simulink model "longitudinal_L1"  (R2023b)
settings: Solver=ode45  StartTime=0.0  StopTime=scn.t_end  MaxStep=0.01  RelTol=1e-3
undefined symbols (not defined in the file): bat, lim, scn, thr, veh
settings Model: Creator=Pol Cruañas  LastModifiedBy=Pol Cruañas

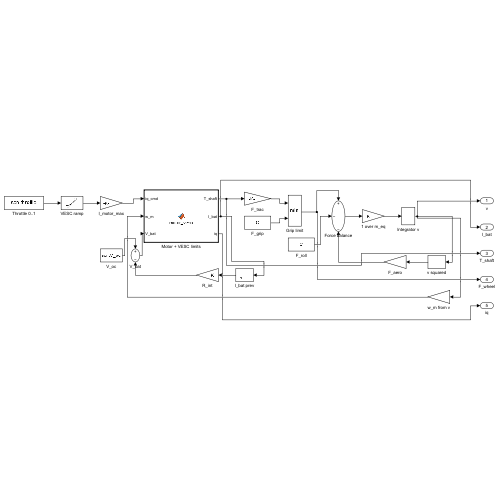
[thumbnail: Simulink's stored preview of the top-level diagram]
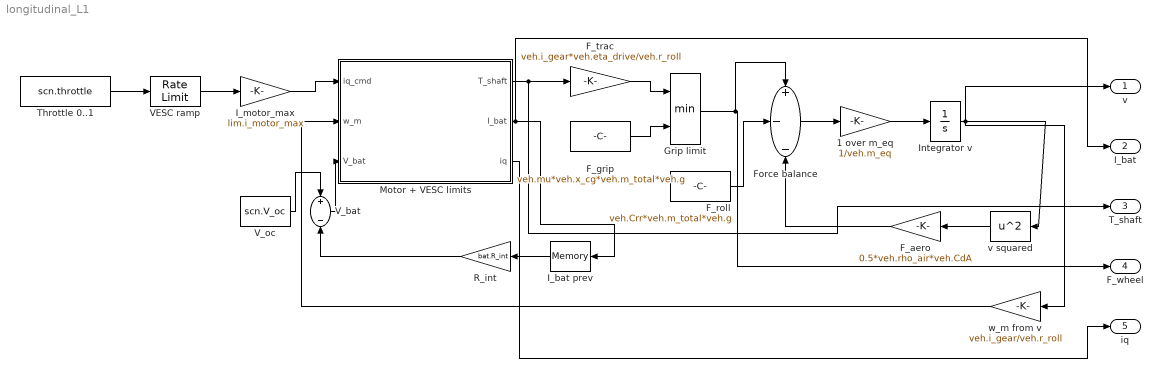
== system longitudinal_L1 ==
  1 over m_eq : Gain  Gain=1/veh.m_eq
  F_aero : Gain  Gain=0.5*veh.rho_air*veh.CdA
  F_grip : Constant  Value=veh.mu*veh.x_cg*veh.m_total*veh.g
  F_roll : Constant  Value=veh.Crr*veh.m_total*veh.g
  F_trac : Gain  Gain=veh.i_gear*veh.eta_drive/veh.r_roll
  Force balance : Sum  Inputs=+--
  Grip limit : MinMax  Inputs=2
  I_bat prev : Memory
  I_motor_max : Gain  Gain=lim.i_motor_max
  Integrator v : Integrator  InitialCondition=scn.v0  LimitOutput=on  LowerSaturationLimit=0
  Motor + VESC limits : MATLAB Function  TreatAsAtomicUnit=on
  R_int : Gain  Gain=bat.R_int
  Throttle 0..1 : FromWorkspace  VariableName=scn.throttle
  VESC ramp : RateLimiter  RisingSlewLimit=1/thr.ramp_time_pos  FallingSlewLimit=-1/thr.ramp_time_neg  SampleTimeMode=inherited
  V_bat : Sum  Inputs=+-
  V_oc : Constant  Value=scn.V_oc
  v squared : Math  Operator=square
  w_m from v : Gain  Gain=veh.i_gear/veh.r_roll
  v : Outport
  I_bat : Outport  Port=2
  T_shaft : Outport  Port=3
  F_wheel : Outport  Port=4
  iq : Outport  Port=5
  wires:
  Throttle 0..1/1 -> VESC ramp/1
  VESC ramp/1 -> I_motor_max/1
  I_motor_max/1 -> Motor + VESC limits/1(iq_cmd)
  w_m from v/1 -> Motor + VESC limits/2(w_m)
  V_bat/1 -> Motor + VESC limits/3(V_bat)
  Motor + VESC limits/1(T_shaft) -> F_trac/1, T_shaft/1
  Motor + VESC limits/2(I_bat) -> I_bat prev/1, I_bat/1
  I_bat prev/1 -> R_int/1
  V_oc/1 -> V_bat/1
  R_int/1 -> V_bat/2
  F_trac/1 -> Grip limit/1
  F_grip/1 -> Grip limit/2
  Grip limit/1 -> Force balance/1, F_wheel/1
  F_roll/1 -> Force balance/2
  F_aero/1 -> Force balance/3
  Force balance/1 -> 1 over m_eq/1
  1 over m_eq/1 -> Integrator v/1
  Integrator v/1 -> v squared/1, w_m from v/1, v/1
  v squared/1 -> F_aero/1
  Motor + VESC limits/3(iq) -> iq/1

== matlab function longitudinal_L1/Motor + VESC limits ==
  data: iq_cmd input; T_shaft output; w_m input; V_bat input; I_bat output; iq output; P parameter
function [T_shaft, I_bat, iq] = motor_vesc(iq_cmd, w_m, V_bat, P)
% Quasi-static PMSM with id = 0 and the three VESC limits on iq.
we = P.p * w_m;                                % electrical speed [rad/s]
Vmax = P.duty_max * V_bat / sqrt(3);           % SVPWM voltage ceiling
% 1) Voltage limit: |v_dq| = Vmax, vd = -we*Lq*iq, vq = R*iq + we*lambda
a  = P.Rs^2 + (we*P.Lq)^2;
bq = 2*P.Rs*we*P.lambda;
c  = (we*P.lambda)^2 - Vmax^2;
disc = bq^2 - 4*a*c;
if disc > 0
    iq_v = (-bq + sqrt(disc)) / (2*a);
else
    iq_v = 0;
end
% 2) Battery-current limit: 1.5*(R*iq^2 + we*lambda*iq) = V_bat*I_bat_max
ab = 1.5*P.Rs;  bb = 1.5*we*P.lambda;  cb = -V_bat*P.i_batt_max;
iq_b = (-bb + sqrt(bb^2 - 4*ab*cb)) / (2*ab);
% 3) Commanded current, then the smallest of the three wins
iq = max(min([iq_cmd, iq_v, iq_b]), 0);
T_em = 1.5 * P.p * P.lambda * iq;
T_drag = P.T_c * (w_m > 1) + P.b * w_m;        % rotor drag, MEASURED C00
T_shaft = T_em - T_drag;
I_bat = 1.5*(P.Rs*iq^2 + we*P.lambda*iq) / V_bat;   % inverter losses ignored
